simulink model "zad2"  (R2022b)
settings: Solver=FixedStepAuto  StartTime=0.0  StopTime=5  FixedStep=0.00001  RelTol=1e-3
model workspace (MAT data in the model file):
  a0 = 1
  a1 = 1
settings Model: Creator=vandm  LastModifiedBy=vandm

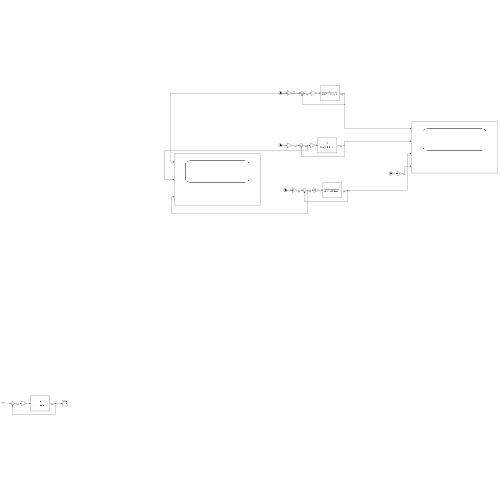
[thumbnail: Simulink's stored preview of the top-level diagram]
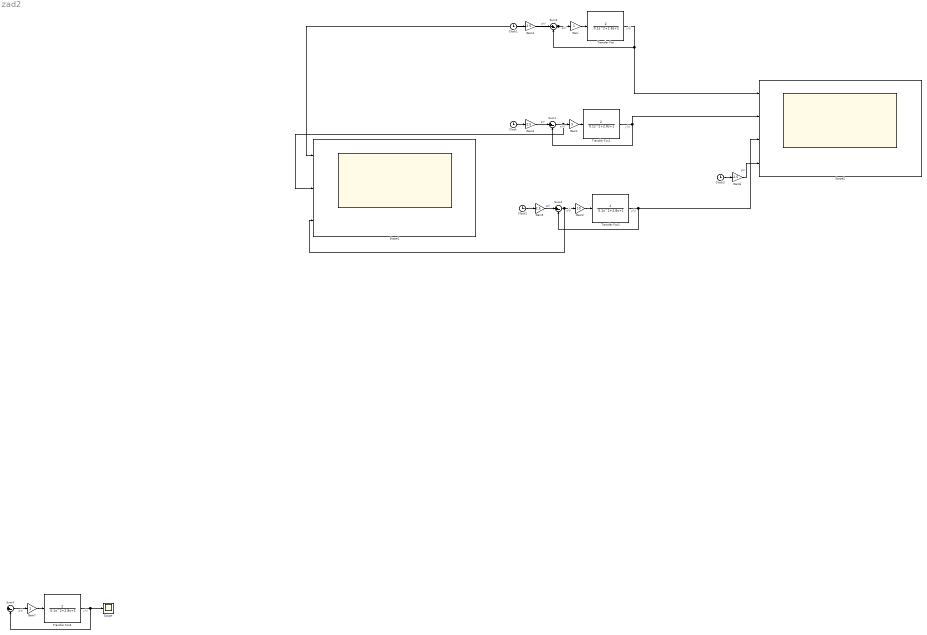
== system zad2 ==
  note: e(t)
  note: y(t)
  note: y(t)
  note: e(t)
  note: y(t)
  note: e(t)
  note: y(t)
  note: e(t)
  Clock{,1..3} (4 alike) : Clock
  Gain : Gain
  Gain1 : Gain  Gain=5
  Gain2 : Gain  Gain=10
  Gain{3..6} (4 alike) : Gain  Gain=2.5
  Gain7 : Gain
  Scope : Scope
  Scope1 : Scope  NumInputPorts=3
  Scope2 : Scope  NumInputPorts=4
  Sum{1..4} (4 alike) : Sum  Inputs=|+-
  Transfer Fcn{,1..3} (4 alike) : TransferFcn  Numerator=[2]  Denominator=[0.1 2.8 1]
  wires:
  Gain4/1 -> Sum2/1  "g(t)"
  Sum2/1 -> Scope1/1, Gain/1
  Gain/1 -> Transfer Fcn/1
  Transfer Fcn/1 -> Scope2/1, Sum2/2
  Sum1/1 -> Scope1/2, Gain1/1
  Gain3/1 -> Sum1/1  "g(t)"
  Gain1/1 -> Transfer Fcn1/1
  Transfer Fcn1/1 -> Scope2/2, Sum1/2
  Transfer Fcn2/1 -> Scope2/3, Sum3/2
  Gain5/1 -> Sum3/1  "g(t)"
  Gain2/1 -> Transfer Fcn2/1
  Sum3/1 -> Scope1/3, Gain2/1
  Gain6/1 -> Scope2/4  "g(t)"
  Clock/1 -> Gain3/1
  Clock1/1 -> Gain4/1
  Clock2/1 -> Gain5/1
  Clock3/1 -> Gain6/1
  Sum4/1 -> Gain7/1
  Gain7/1 -> Transfer Fcn3/1
  Transfer Fcn3/1 -> Scope/1, Sum4/2
  ? -> Sum4/1  "g(t)"
